simulink model "PE_Boost"  (R2025a)
settings: Solver=VariableStepAuto  StartTime=0.0  StopTime=1  FixedStep=1e-6  MaxStep=1e-6  RelTol=1e-4
libraries: spsDiodeLib x5, spsSeriesRLCBranchLib x3, spsCurrentMeasurementLib x2, spsACVoltageSourceLib x1, spsMosfetLib x1, eePwmGenerator x1, spsVoltageMeasurementLib x1, sps_lib x1
settings Model: Creator=abhis  LastModifiedBy=abhis

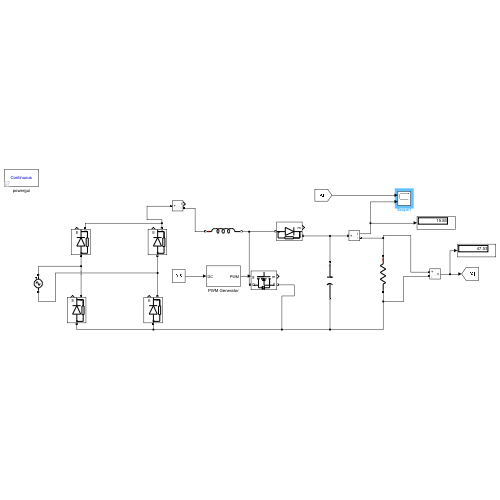
[thumbnail: Simulink's stored preview of the top-level diagram]
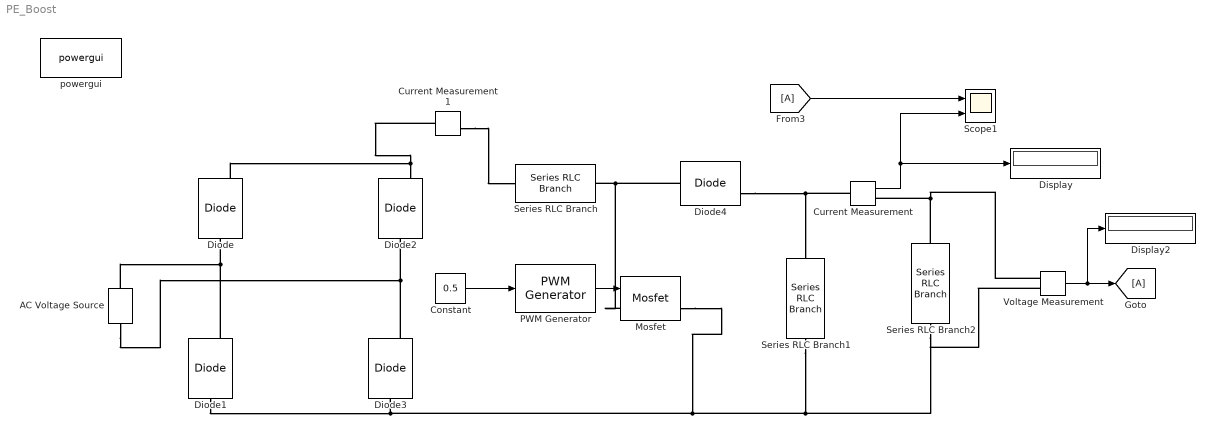
== system PE_Boost ==
  AC Voltage Source : spsACVoltageSourceLib/AC Voltage Source  Amplitude=30  Phase=0  Frequency=50  SampleTime=0  Measurements=None  BusType=swing  Pref=10e3  Qref=0  Qmin=-inf  Qmax=+inf
  Constant : Constant  Value=0.5
  Current Measurement : spsCurrentMeasurementLib/Current Measurement  PhasorSimulation=off  OutputType=Complex  PSBequivalent=0
  Current Measurement1 : spsCurrentMeasurementLib/Current Measurement  PhasorSimulation=off  OutputType=Complex  PSBequivalent=0
  Diode{,1..4} (5 alike) : spsDiodeLib/Diode  Ron=0.001  Lon=0  Vf=0.8  IC=0  UseSnubber=0  Rs=500  Cs=250e-9  Measurements=on
  Display : Display
  Display2 : Display
  From3 : From
  Goto : Goto
  Mosfet : spsMosfetLib/Mosfet  Ron=0.1  Lon=0  Rd=0.01  Vfd=0  IC=0  Rs=1e5  Cs=inf  Measurements=on
  PWM Generator : eePwmGenerator/PWM Generator  CarrCount=Up  Tper=0.001  Tdelay=0  Ts=5e-5
  Scope1 : Scope  NumInputPorts=2
      settings: ActiveDisplayYMinimum=3.0745374311738018  ActiveDisplayYMaximum=52.104537788845533
  Series RLC Branch : spsSeriesRLCBranchLib/Series RLC Branch  LConnTagsString=__new0  RConnTagsString=__new0  BranchType=L  Resistance=1  Inductance=56e-6  SetiL0=off  InitialCurrent=0  Capacitance=1e-6  Setx0=off  InitialVoltage=0  Measurements=None
  Series RLC Branch1 : spsSeriesRLCBranchLib/Series RLC Branch  LConnTagsString=__new0  RConnTagsString=__new0  BranchType=C  Resistance=1  Inductance=1e-3  SetiL0=off  InitialCurrent=0  Capacitance=0.120  Setx0=off  InitialVoltage=0  Measurements=None
  Series RLC Branch2 : spsSeriesRLCBranchLib/Series RLC Branch  LConnTagsString=__new0  RConnTagsString=__new0  BranchType=R  Resistance=3  Inductance=1e-3  SetiL0=off  InitialCurrent=0  Capacitance=1e-6  Setx0=off  InitialVoltage=0  Measurements=None
  Voltage Measurement : spsVoltageMeasurementLib/Voltage Measurement  PhasorSimulation=off  OutputType=Complex  PSBequivalent=0
  powergui : sps_lib/powergui  Priority=1  SimulationMode=Continuous  SampleTime=50e-6  frequency=60  Iterations=50  frequencyindice=50  Pbase=100e6  ErrMax=1e-4  UnitsV=kV  UnitsW=MW  buscounter=0  FunctionMessages=off  echomessages=off  EnableUseOfTLC=off  CurrentSourceSwitches=off  DisableSnubberDevices=off  DisableRonSwitches=off  DisableVfSwitches=off  DisplayEquations=off  AutomaticDiscreteSolvers=off  SolverType=Tustin/Backward Euler (TBE)  Interpol=off  ExternalGateDelay=off  methode=off  Ts=100  x0status=blocks  SPID=on  SwTol=0  HookPort=off  NonlinearTolerance=1e-4  nMaxIteration=100  ContinueOnMaxIteration=off  RestoreLinks=warning  ResistiveCurrentMeasurement=off  Frange=[0:2:500]  Ylog=off  Xlog=on  ShowGrid=off  save=off  variable=ZData  structure=0  ZoomFFT=off  StartTime=0.0  cycles=1  DisplayStyle=1  fundamental=60  FreqAxis=off  MaxFrequency=1000  frequencyindicesteady=1  RmsSteady=1  display=off
  wires:
  PWM Generator/1 -> Mosfet/1
  Voltage Measurement/1 -> Display2/1, Goto/1
  From3/1 -> Scope1/1
  Current Measurement/1 -> Scope1/2, Display/1
  Constant/1 -> PWM Generator/1
  connections:
  Diode1/RConn1 -- AC Voltage Source/RConn1 -- Diode/LConn1
  Diode3/RConn1 -- AC Voltage Source/LConn1 -- Diode2/LConn1
  Diode1/LConn1 -- Series RLC Branch1/RConn1 -- Voltage Measurement/LConn2 -- Series RLC Branch2/RConn1 -- Mosfet/RConn1 -- Diode3/LConn1
  Diode/RConn1 -- Current Measurement1/LConn1 -- Diode2/RConn1
  Mosfet/LConn1 -- Diode4/LConn1 -- Series RLC Branch/RConn1
  Diode4/RConn1 -- Current Measurement/LConn1 -- Series RLC Branch1/LConn1
  Series RLC Branch2/LConn1 -- Voltage Measurement/LConn1 -- Current Measurement/RConn1
  Current Measurement1/RConn1 -- Series RLC Branch/LConn1
